simulink model "trail5freqchangeBandF_analog_uart1"  (Simulink 7.0)
settings: Solver=FixedStepDiscrete  StartTime=0.0  StopTime=10  FixedStep=0.001  RelTol=1e-3
libraries: dsPICdrivers x12, simulink x2
settings Model: Creator=Chandupotluri  LastModifiedBy=ProjectG
settings OptimizationCC: OptimizeModelRefInitCode=on  LifeSpan=1
settings HardwareCC: TargetHWDeviceType=32-bit Generic
settings RTWCC: SystemTargetFile=pic32.tlc  TemplateMakefile=pic32_gcc.tmf  PostCodeGenCommand=dsPIC_Compile()  Description=Embedded Target for Microchip dsPIC (real-time)  ProcessScript=pic32_make_rtw_hook
settings CodeAppCC: IgnoreCustomStorageClasses=off
settings STFCustomTargetCC: GenFloatMathFcnCalls=ANSI_C  ModelReferenceCompliant=off  IncludeMdlTerminateFcn=off  CombineOutputUpdateFcns=on  SuppressErrorStatus=on  ERTCustomFileBanners=on  SupportContinuousTime=off  SupportNonInlinedSFcns=off  SystemTargetFile=pic32.tlc
settings ERTTargetCC: GenFloatMathFcnCalls=ANSI_C  ModelReferenceCompliant=off  CompOptLevelCompliant=off  IncludeMdlTerminateFcn=off  SuppressErrorStatus=on  ModelStepFunctionPrototypeControlCompliant=off  InlinedParameterPlacement=NonHierarchical  ERTSrcFileBannerTemplate=dsPIC_code_template.cgt  ERTHdrFileBannerTemplate=dsPIC_code_template.cgt  ERTDataSrcFileTemplate=dsPIC_code_template.cgt  ERTDataHdrFileTemplate=dsPIC_code_template.cgt  ERTCustomFileTemplate=dsPIC_main.tlc
settings CustomProperty: DataType=string  Value=C:\PROGRA~1\MATLAB\R2007b\bin\win32\gmake

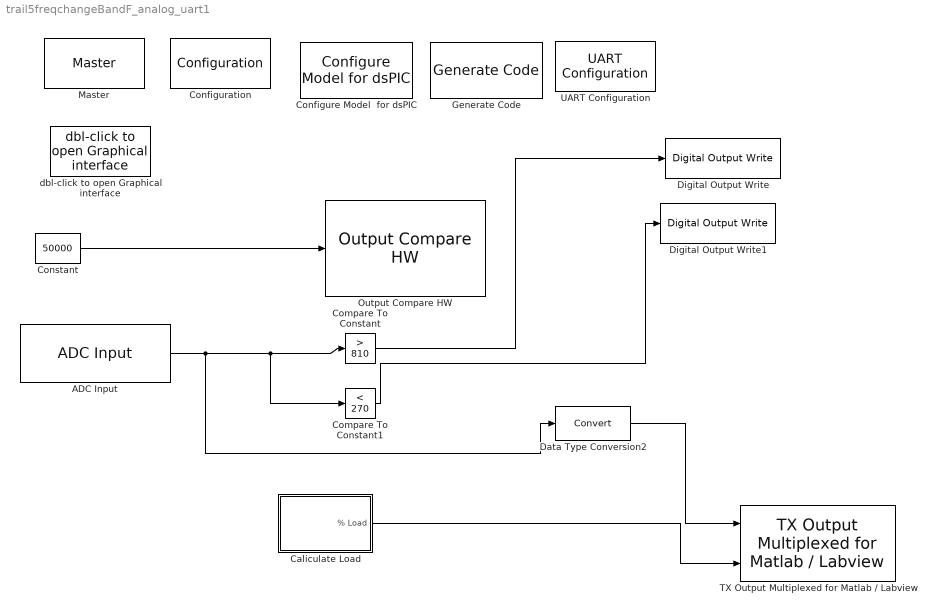
== system trail5freqchangeBandF_analog_uart1 ==
  ADC Input : dsPICdrivers/Peripheral I//O/ADC Input  Tag=dsPIC_ADC  Priority=5  ADC_TYPE=10 bits  ADC_MODE=Continuous sampling & get last channel value  NbrSampleStep=1  VoltRefpopup="AVdd  -  AVss"  OutFormatBitspopup=0000 00dd dddd dddd : Integer  InterruptPriority=6  ANCHANNELS=[2]  MaxName=ANmax = 1023  Rin=1e2  ADCS=11  SAMC=1  Temperature=25  DMAChannel=1  SampleTime=0.01  Status="OK  |  Tsmp=1.600e-007 |  T/Channel=2.080e-006 |  Tall=2.080e-006"  SSRC=auto convert
  Caliculate Load : Subsystem
  Compare To Constant : simulink/Logic and Bit Operations/Compare To Constant  SystemSampleTime=-1  relop=>  const=810  LogicOutDataTypeMode=boolean  ZeroCross=off
  Compare To Constant1 : simulink/Logic and Bit Operations/Compare To Constant  SystemSampleTime=-1  relop=<  const=270  LogicOutDataTypeMode=boolean  ZeroCross=off
  Configuration : dsPICdrivers/Configuration  SystemSampleTime=-1  double64=off
  Configure Model  for dsPIC : dsPICdrivers/Simulink Configuration/Configure Model  for dsPIC
  Constant : Constant  Value=50000  OutMin=[0]  OutMax=[65000]  OutDataTypeMode=uint16  OutDataType=sfix(16)  OutScaling=2^0  SampleTime=0.01
  Data Type Conversion2 : DataTypeConversion  OutDataTypeMode=uint16  OutDataType=sfix(16)  OutScaling=2^0
  Digital Output Write : dsPICdrivers/Digital I//O/Digital Output Write  Tag=dsPIC_Digital_Output  Priority=5  PORT=C  Pin=[1]  Simultaneous=off  OrderingInOutPopup=None
  Digital Output Write1 : dsPICdrivers/Digital I//O/Digital Output Write  Tag=dsPIC_Digital_Output  Priority=5  PORT=C  Pin=[2]  Simultaneous=off  OrderingInOutPopup=None
  Generate Code : dsPICdrivers/Simulink Configuration/Generate Code
  Master : dsPICdrivers/Master  Tag=dsPIC_MASTER  Priority=1  TimeStepType=Timer1  picType=32MX360F512L  fcy=37500000  Quartz_33f=2.5e6  PLLActive_33f=on  fcyDesired_33f=40000000  tmr1="[1  37499  0]"  tmr1Info="Time Step : 0.001  ;   Error : 0%  PR1=37499"  tmr2345="[64   0   0   0]"  tmr2345cfg=[-1 -1 -1 -1]  IOautoConf=on  typePort="[ 0   0   0   0   0   0   0   0   0   0   0   0   0   0   0   0   0   0   8   0   0   0   0   0   0   0   0   0   0   0   0   0   0  10  10   0   0   0   0   0   0   0   0   0   0   0   0   0   0   0   0   0  24   0   0   0   0   0   0   0   0   0   0   0   0   0   0   0   0   0   0   0   0   0   0   0   0   0   0   0   0   0   0   0   4   5   0   0   0   0   0   0   0   0   0   0   0   0   0   0   0   0   0   0   0   0   0   0   0   0   0   0 ]"  TRIS="[ 65535  65535  65529  65519  65535  65535  65535 ]"  ADPCFG=0  MasterBusyPort=None  MasterOverloadPort=None  FOSC=Quartz (XT - HS)  ClockSwitchMonitor=Both disabled  TempProtection_33f=TEMP_ON  FPBOR=<empty>  PWRT=disable  MCLR=<empty>  PowerSave=off  OverrideFcy=off  NewFcy=1e6  PR2345="[58593  65535  65535  65535]"
  Output Compare HW : dsPICdrivers/Peripheral I//O/Output Compare HW  Tag=dsPIC_OC_HW_out  Priority=5  OC_Mode=PWM duty cycle (robust)  Timer=2  CHANNEL=[5]  Channel_UP_Down_Periode=[5]  PeriodeInput=off  MaxChannel=0.1  MaxName=' OCmax '  Precision=[15.8385]  Status=OK  SafeMarge=[0]  PortLetter=[68]  PortNumber=[4]  MaxValues=[58593]  NPORTS=1
  TX Output Multiplexed for Matlab / Labview : dsPICdrivers/Serial PORT/TX Output Multiplexed for Matlab // Labview  Tag=dsPIC_TX_Multiplexed  Priority=5  UART=2  CleverSpreadingChk=on  CleverSpreading=1  CHANNEL=[0 1]  CHANNELBLOCKED=[]  CHANNELBLOCKED_BITEWISE=0  Status=OK
  UART Configuration : dsPICdrivers/Serial PORT/UART Configuration  Tag=dsPIC_config_UART  Priority=2  UART=2  proposed_BAUD=115200  ALT_TX_RX=off  InterruptTxWhen=When Transmit Buffer is empty  TXInterruptPri=1  TxBufferSize=32  TXEN=on  InterruptRxWhen=When Receive Buffer is full (contain 4 characters)  RXInterruptPri=2  RxBufferSize=32  BAUD=38400  UxBRG=60  Info="UxBRG = 19   ||  Real Baud : 117188   ||  % error : 1.7253  ||  max 11.7188 Bytes / Step"  RealBaud=0
  dbl-click to open Graphical interface : dsPICdrivers/Serial PORT/dbl-click to open Graphical interface  SystemSampleTime=-1  Nothing=0
  wires:
  Constant/1 -> Output Compare HW/1
  Data Type Conversion2/1 -> TX Output Multiplexed for Matlab / Labview/1
  Caliculate Load/1(% Load) -> TX Output Multiplexed for Matlab / Labview/2
  ADC Input/1 -> Compare To Constant/1, Compare To Constant1/1, Data Type Conversion2/1
  Compare To Constant1/1 -> Digital Output Write1/1
  Compare To Constant/1 -> Digital Output Write/1

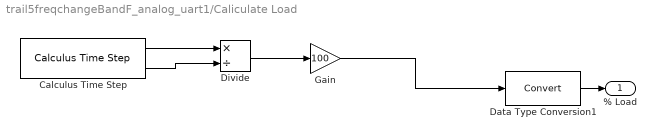
== system trail5freqchangeBandF_analog_uart1/Caliculate Load ==
  Calculus Time Step : dsPICdrivers/OTHERS/Calculus Time Step  Tag=dsPIC_CalculusTimeStep  SampleTime=0.01  PR1chk=on
  Data Type Conversion1 : DataTypeConversion  OutDataTypeMode=uint16  OutDataType=sfix(16)  OutScaling=2^0
  Divide : Product  Inputs=*/  OutDataType=sfix(16)  OutScaling=2^-10
  Gain : Gain  Gain=100  ParameterDataType=sfix(16)  ParameterScaling=2^0  OutDataType=sfix(16)  OutScaling=2^0
  % Load : Outport
  wires:
  Calculus Time Step/1 -> Divide/1
  Calculus Time Step/2 -> Divide/2
  Divide/1 -> Gain/1
  Gain/1 -> Data Type Conversion1/1
  Data Type Conversion1/1 -> % Load/1
